simulink model "Factory_Physics_Model"  (R2024b)
settings: Solver=ode4  StartTime=0  StopTime=45  FixedStep=0.0005  RelTol=1e-3
model workspace (MAT data in the model file):
  FACTORY_EXT_CMD = 0
settings Model: Creator=shash  LastModifiedBy=shash
settings ModelReferenceCC: ModelReferenceNumInstancesAllowed=Single

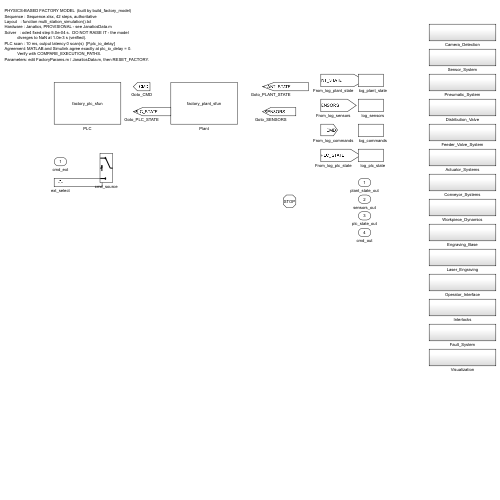
[thumbnail: Simulink's stored preview of the top-level diagram]
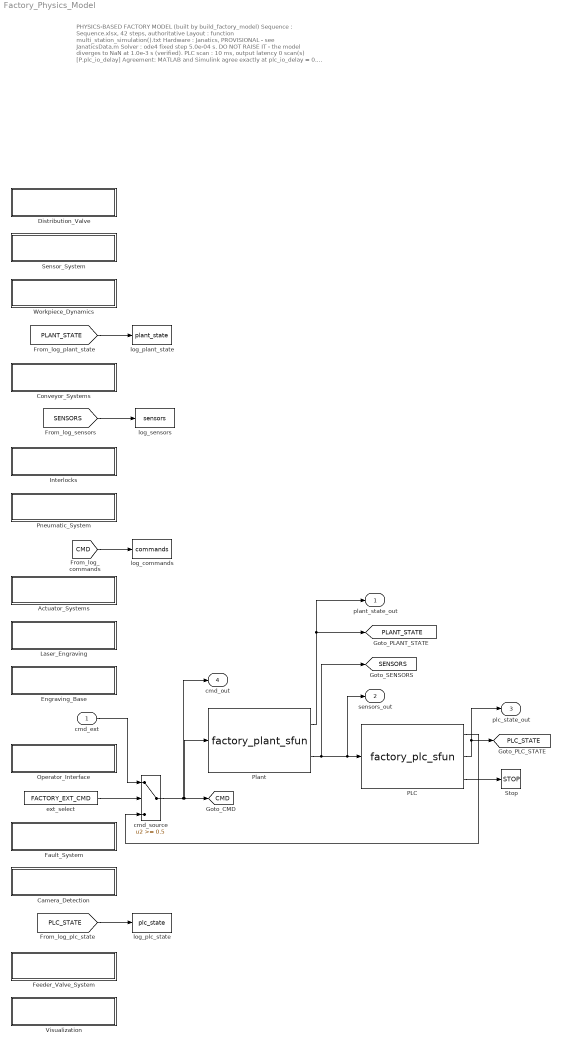
== system Factory_Physics_Model ==
  note: PHYSICS-BASED FACTORY MODEL  (built by build_factory_model)
      | Sequence : Sequence.xlsx, 42 steps, authoritative
      | Layout   : function multi_station_simulation().txt
      | Hardware : Janatics, PROVISIONAL - see JanaticsData.m
      | Solver   : ode4 fixed step 5.0e-04 s.  DO NOT RAISE IT - the model
      |            diverges to NaN at 1.0e-3 s (verified).
      | PLC scan : 10 ms, output latency 0 scan(s)  [P.plc_io_delay]
      | Agreement: MATLAB and Simulink agree exactly at plc_io_delay = 0.
      |            Verify with COMPARE_EXECUTION_PATHS.
      | Parameters: edit FactoryParams.m / JanaticsData.m, then RESET_FACTORY.
  cmd_ext : Inport  PortDimensions=22
  Actuator_Systems : Subsystem
  Camera_Detection : Subsystem
  Conveyor_Systems : Subsystem
  Distribution_Valve : Subsystem
  Engraving_Base : Subsystem
  Fault_System : Subsystem
  Feeder_Valve_System : Subsystem
  Interlocks : Subsystem
  Laser_Engraving : Subsystem
  Operator_Interface : Subsystem
  PLC : M-S-Function  FunctionName=factory_plc_sfun
  Plant : M-S-Function  FunctionName=factory_plant_sfun
  Pneumatic_System : Subsystem
  Sensor_System : Subsystem
  Stop : Stop
  Visualization : Subsystem
  Workpiece_Dynamics : Subsystem
  cmd_source : Switch  Threshold=0.5
  ext_select : Constant  Value=FACTORY_EXT_CMD
  log_commands : ToWorkspace  VariableName=commands  SaveFormat=Structure With Time
      settings: Decimation=20
  log_plant_state : ToWorkspace  VariableName=plant_state  SaveFormat=Structure With Time
      settings: Decimation=20
  log_plc_state : ToWorkspace  VariableName=plc_state  SaveFormat=Structure With Time
      settings: Decimation=20
  log_sensors : ToWorkspace  VariableName=sensors  SaveFormat=Structure With Time
      settings: Decimation=20
  plant_state_out : Outport
  sensors_out : Outport  Port=2
  plc_state_out : Outport  Port=3
  cmd_out : Outport  Port=4
  tag scope: CMD=global, PLANT_STATE=global, PLC_STATE=global, SENSORS=global
  wires:
  [PLANT_STATE] -> log_plant_state/1
  [SENSORS] -> log_sensors/1
  [CMD] -> log_commands/1
  Plant/1 -> [PLANT_STATE], plant_state_out/1
  [PLC_STATE] -> log_plc_state/1
  PLC/3 -> Stop/1
  PLC/1 -> cmd_source/3
  cmd_ext/1 -> cmd_source/1
  cmd_source/1 -> Plant/1, [CMD], cmd_out/1
  ext_select/1 -> cmd_source/2
  PLC/2 -> [PLC_STATE], plc_state_out/1
  Plant/2 -> PLC/1, sensors_out/1, [SENSORS]

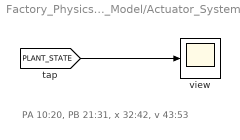
== system Factory_Physics_Model/Actuator_Systems ==
  note: PA 10:20, PB 21:31, x 32:42, v 43:53
  view : Scope
  wires:
  [PLANT_STATE] -> view/1

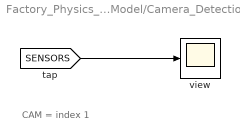
== system Factory_Physics_Model/Camera_Detection ==
  note: CAM = index 1
  view : Scope
  wires:
  [SENSORS] -> view/1

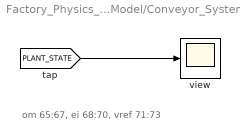
== system Factory_Physics_Model/Conveyor_Systems ==
  note: om 65:67, ei 68:70, vref 71:73
  view : Scope
  wires:
  [PLANT_STATE] -> view/1

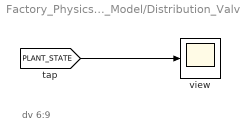
== system Factory_Physics_Model/Distribution_Valve ==
  note: dv 6:9
  view : Scope
  wires:
  [PLANT_STATE] -> view/1

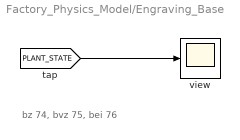
== system Factory_Physics_Model/Engraving_Base ==
  note: bz 74, bvz 75, bei 76
  view : Scope
  wires:
  [PLANT_STATE] -> view/1

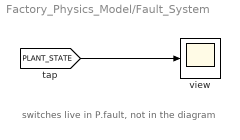
== system Factory_Physics_Model/Fault_System ==
  note: switches live in P.fault, not in the diagram
  view : Scope
  wires:
  [PLANT_STATE] -> view/1

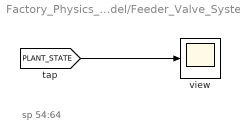
== system Factory_Physics_Model/Feeder_Valve_System ==
  note: sp 54:64
  view : Scope
  wires:
  [PLANT_STATE] -> view/1

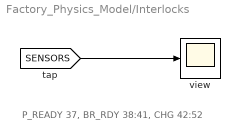
== system Factory_Physics_Model/Interlocks ==
  note: P_READY 37, BR_RDY 38:41, CHG 42:52
  view : Scope
  wires:
  [SENSORS] -> view/1

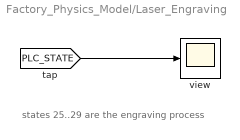
== system Factory_Physics_Model/Laser_Engraving ==
  note: states 25..29 are the engraving process
  view : Scope
  wires:
  [PLC_STATE] -> view/1

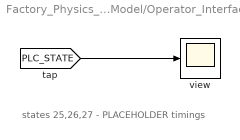
== system Factory_Physics_Model/Operator_Interface ==
  note: states 25,26,27 - PLACEHOLDER timings
  view : Scope
  wires:
  [PLC_STATE] -> view/1

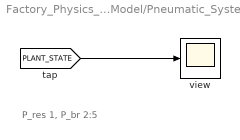
== system Factory_Physics_Model/Pneumatic_System ==
  note: P_res 1, P_br 2:5
  view : Scope
  wires:
  [PLANT_STATE] -> view/1

== system Factory_Physics_Model/Sensor_System ==
  note: PX 2:11, EXT 12:22, RET 23:33, HS_TOP 34, HS_BOT 35
  view : Scope
  wires:
  [SENSORS] -> view/1

== system Factory_Physics_Model/Visualization ==
  note: use visualize_factory(LOG) from MATLAB
  view : Scope
  wires:
  [PLANT_STATE] -> view/1

== system Factory_Physics_Model/Workpiece_Dynamics ==
  note: bx 77, by 78, bvx 79, bvy 80
  view : Scope
  wires:
  [PLANT_STATE] -> view/1
